simulink library "Contact_Forces_Lib"  (R2025b)
settings: Solver=ode45  StartTime=0.0  StopTime=10.0  RelTol=1e-3  EnableMultiTasking=on
undefined symbols (not defined in the file or in its folder): b_contact, custom_param_1, custom_param_2, Extr_Data_Ring, k_contact, l_cone, length_cylinder, length_tube, mu_kinetic, mu_static, pen_exponent, pen_full_damp_F, rad_s_cone, radius_cylinder, radius_tube, v_thr, X, Y, Z
libraries: nesl_utility x197, sm_lib x115, $bdroot x72, simulink x20, fl_lib x4
(part 7 of 12)

== system Contact_Forces_Lib/3D/Sphere in Sphere Force/Sensing ==
  Divide : Product  Inputs=*/
  Mux : Mux  Inputs=3
  Mux1 : Mux  Inputs=3
  Mux2 : Mux  Inputs=3
  PS-Simulink Converter{2..4,7..15} (12 alike) : nesl_utility/PS-Simulink Converter  PhysicalDomain=network_engine_domain  SubClassName=ps_output  LeftPortType=input  RightPortType=output  PseudoPeriodic=off  Frequencies=[]  VectorFormat=1-D array  Unit=1  AffineConversion=off
  Transform Sensor : sm_lib/Frames and Transforms/Transform Sensor  MeasurementFrame=Base  RotationSequence=XYX  SenseAngle=off  SenseAxis=off  SenseQ=off  SenseR=on  SenseRotationSequence=off  SenseOmegaX=on  SenseOmegaY=on  SenseOmegaZ=on  SenseOmega=off  SenseQDot=off  SenseRDot=off  SenseRotationSequenceDot=off  SenseAlphaX=off  SenseAlphaY=off  SenseAlphaZ=off  SenseAlpha=off  SenseQDDot=off  SenseRDDot=off  SenseX=on  SenseY=on  SenseZ=on  SenseXYZ=off  SenseRad=off  SenseAzim=off  SenseDist=on  SenseInc=off  SenseXDot=on  SenseYDot=on  SenseZDot=on  SenseXYZDot=off  SenseRadDot=off  SenseAzimDot=off  SenseDistDot=on  SenseIncDot=off  SenseXDDot=off  SenseYDDot=off  SenseZDDot=off  SenseXYZDDot=off  SenseRadDDot=off  SenseAzimDDot=off  SenseDistDDot=off  SenseIncDDot=off
  F : PMIOPort  Side=Left
  B : PMIOPort  Port=2  Side=Left
  R : Outport  VectorParamsAs1DForOutWhenUnconnected=off
  dst : Outport  Port=2  VectorParamsAs1DForOutWhenUnconnected=off
  vdst : Outport  Port=3  VectorParamsAs1DForOutWhenUnconnected=off
  dvect : Outport  Port=4  VectorParamsAs1DForOutWhenUnconnected=off
  v : Outport  Port=5  VectorParamsAs1DForOutWhenUnconnected=off
  w : Outport  Port=6  VectorParamsAs1DForOutWhenUnconnected=off
  wires:
  PS-Simulink Converter2/1 -> R/1
  PS-Simulink Converter7/1 -> Divide/2, dst/1
  PS-Simulink Converter8/1 -> vdst/1
  PS-Simulink Converter11/1 -> Mux/3
  PS-Simulink Converter10/1 -> Mux/2
  PS-Simulink Converter9/1 -> Mux/1
  Mux/1 -> Divide/1
  Divide/1 -> dvect/1
  PS-Simulink Converter3/1 -> Mux1/1
  PS-Simulink Converter4/1 -> Mux1/2
  PS-Simulink Converter12/1 -> Mux1/3
  Mux1/1 -> w/1
  PS-Simulink Converter14/1 -> Mux2/2
  PS-Simulink Converter15/1 -> Mux2/3
  PS-Simulink Converter13/1 -> Mux2/1
  Mux2/1 -> v/1
  connections:
  Transform Sensor/RConn1 -- F/RConn1
  Transform Sensor/LConn1 -- B/RConn1
  Transform Sensor/RConn2 -- PS-Simulink Converter2/LConn1
  Transform Sensor/RConn3 -- PS-Simulink Converter3/LConn1
  PS-Simulink Converter4/LConn1 -- Transform Sensor/RConn4
  PS-Simulink Converter8/LConn1 -- Transform Sensor/RConn13
  PS-Simulink Converter7/LConn1 -- Transform Sensor/RConn9
  Transform Sensor/RConn8 -- PS-Simulink Converter11/LConn1
  Transform Sensor/RConn7 -- PS-Simulink Converter10/LConn1
  Transform Sensor/RConn6 -- PS-Simulink Converter9/LConn1
  PS-Simulink Converter12/LConn1 -- Transform Sensor/RConn5
  PS-Simulink Converter13/LConn1 -- Transform Sensor/RConn10
  PS-Simulink Converter14/LConn1 -- Transform Sensor/RConn11
  PS-Simulink Converter15/LConn1 -- Transform Sensor/RConn12

== system Contact_Forces_Lib/3D/Sphere to Cone Force/Check Active ==
  z : Inport
  azm : Inport  Port=2
  Check Active Range : Subsystem
  Data Type Conversion : DataTypeConversion  SaturateOnIntegerOverflow=off  RndMeth=Floor
  In Tube : Subsystem
  Logical Operator : Logic  AllPortsSameDT=off  OutDataTypeStr=boolean
  En : Outport  VectorParamsAs1DForOutWhenUnconnected=off
  wires:
  Data Type Conversion/1 -> En/1
  In Tube/1(En) -> Logical Operator/1
  azm/1 -> Check Active Range/1(azm)
  z/1 -> In Tube/1(z)
  Check Active Range/1(En) -> Logical Operator/2
  Logical Operator/1 -> Data Type Conversion/1

== system Contact_Forces_Lib/3D/Sphere to Cone Force/Demux ==
  Frc : Inport
  Cone Forces : Scope  NumInputPorts=6
      settings: ActiveDisplayYMinimum=-7.50703109533E+6  ActiveDisplayYMaximum=872315.20608
  Demux : Demux  Outputs=8
  Demux1 : Demux  Outputs=3
  Demux2 : Demux  Outputs=3
  Simulink-PS Converter{,1..7} (8 alike) : nesl_utility/Simulink-PS Converter  PhysicalDomain=network_engine_domain  SubClassName=ps_input  LeftPortType=input  RightPortType=output  PseudoPeriodic=off  Frequencies=[]  NoiseDistribution=none  NoiseParameters=[]  Unit=1  AffineConversion=off  FilteringAndDerivatives=zero  SimscapeFilterOrder=1  InputFilterTimeConstant=0.005  UdotUserProvided=1
  Sphere Forces : Scope  NumInputPorts=6
      settings: ActiveDisplayYMinimum=-114928.22843  ActiveDisplayYMaximum=94591.09777
  FxF : PMIOPort  Side=Right
  FyF : PMIOPort  Port=2  Side=Right
  FzF : PMIOPort  Port=3  Side=Right
  TF : PMIOPort  Port=4  Side=Right
  FxB : PMIOPort  Port=5  Side=Right
  FyB : PMIOPort  Port=6  Side=Right
  FzB : PMIOPort  Port=7  Side=Right
  TB : PMIOPort  Port=8  Side=Right
  wires:
  Demux2/3 -> Cone Forces/6  "Tz"
  Demux2/2 -> Cone Forces/5  "Ty"
  Demux2/1 -> Cone Forces/4  "Tx"
  Demux1/3 -> Sphere Forces/6  "Tz"
  Demux1/2 -> Sphere Forces/5  "Ty"
  Demux1/1 -> Sphere Forces/4  "Tx"
  Frc/1 -> Demux/1
  Demux/1 -> Sphere Forces/1, Simulink-PS Converter/1  "Fx"
  Demux/2 -> Sphere Forces/2, Simulink-PS Converter1/1  "Fy"
  Demux/4 -> Simulink-PS Converter2/1, Demux1/1
  Demux/3 -> Simulink-PS Converter6/1, Sphere Forces/3  "Fz"
  Demux/8 -> Simulink-PS Converter5/1, Demux2/1
  Demux/5 -> Simulink-PS Converter3/1, Cone Forces/1  "Fx"
  Demux/6 -> Simulink-PS Converter4/1, Cone Forces/2  "Fy"
  Demux/7 -> Simulink-PS Converter7/1, Cone Forces/3  "Fz"
  connections:
  Simulink-PS Converter2/RConn1 -- TF/RConn1
  Simulink-PS Converter4/RConn1 -- FyB/RConn1
  Simulink-PS Converter3/RConn1 -- FxB/RConn1
  Simulink-PS Converter5/RConn1 -- TB/RConn1
  Simulink-PS Converter/RConn1 -- FxF/RConn1
  Simulink-PS Converter1/RConn1 -- FyF/RConn1
  Simulink-PS Converter6/RConn1 -- FzF/RConn1
  Simulink-PS Converter7/RConn1 -- FzB/RConn1

== system Contact_Forces_Lib/3D/Sphere to Cone Force/Forces ==
  z : Inport
  rad : Inport  Port=2
  vrad : Inport  Port=3
  azm : Inport  Port=4
  vazm : Inport  Port=5
  vzf : Inport  Port=6
  wzf : Inport  Port=7
  R : Inport  Port=8
  wxf : Inport  Port=9
  wyf : Inport  Port=10
  vazmx : Inport  Port=11
  vazmy : Inport  Port=12
  Action Port : ActionPort
  Bus Creator : BusCreator  Inputs=6
  Calculate Penetration : Subsystem
  Ff : Subsystem
  Fn : Subsystem
  Force Law : $bdroot/Force Law  SystemSampleTime=-1  LabelModeActiveChoice=Linear  VariantActivationTime=update diagram  EmptyChoice=off  PassThrough=off  PassThroughVariantControl=(default)  EmptyChoiceVariantControl=(default)  AllowFlexibleInterface=on  Latency=0  AutoFrameSizeCalculation=off
  Gain : Gain  Gain=-1
  Mux : Mux  Inputs=8
  Product : Product
  Sum : Subsystem
  Sum1 : Sum  Inputs=+-
  Frc : Outport  VectorParamsAs1DForOutWhenUnconnected=off
  Out : Outport  Port=2  InitialOutput=[0]  VectorParamsAs1DForOutWhenUnconnected=off
  wires:
  vazmy/1 -> Ff/14(vazmy)
  vazmx/1 -> Ff/13(vazmx)
  wyf/1 -> Ff/12(wyf)
  wxf/1 -> Ff/11(wxf)
  Gain/1 -> Ff/1(Fn)
  vazm/1 -> Ff/5(vazm)
  wzf/1 -> Ff/6(wzf)
  Fn/6(FzConB) -> Sum/6(FnzConB)
  Ff/8(TConB) -> Sum/16(TConB)
  Ff/7(TSphF) -> Sum/15(TzSphF)
  Ff/6(FzConB) -> Sum/14(FfzConB)
  Ff/5(FyConB) -> Sum/13(FfyConB)
  Ff/4(FxConB) -> Sum/12(FfxConB)
  Ff/3(FzSphF) -> Sum/11(FfzSphF)
  Ff/2(FySphF) -> Sum/10(FfySphF)
  Ff/1(FxSphF) -> Sum/9(FfxSphF)
  Fn/8(TyConB) -> Sum/8(TnyConB)
  Fn/7(TxConB) -> Sum/7(TnxConB)
  Fn/5(FyConB) -> Sum/5(FnyConB)
  Fn/4(FxConB) -> Sum/4(FnxConB)
  Fn/3(FZSphF) -> Sum/3(FnzSphF)
  Fn/1(FxSphF) -> Sum/1(FnxSphF)
  Fn/2(FySphF) -> Sum/2(FnySphF)
  z/1 -> Fn/2(z), Ff/2(z), Calculate Penetration/3(z)
  Bus Creator/1 -> Out/1
  Force Law/1 -> Bus Creator/4, Sum1/1  "Spr Force"
  Calculate Penetration/3(Pen Vel) -> Bus Creator/1, Force Law/2  "Penetration Vel"
  vrad/1 -> Calculate Penetration/2(vrad), Ff/9(vrad)
  rad/1 -> Calculate Penetration/1(rad), Ff/8(rad), Fn/3(rad)
  Product/1 -> Bus Creator/5, Gain/1, Fn/1(Fn)  "Normal Force"
  Calculate Penetration/2(Pen) -> Force Law/1, Ff/7(Pen), Bus Creator/2  "Penetration"
  Calculate Penetration/1(sign) -> Product/1
  Force Law/2 -> Bus Creator/3, Sum1/2  "Damp Force"
  Sum1/1 -> Product/2
  R/1 -> Fn/4(R), Ff/3(R)
  azm/1 -> Fn/5(azm), Ff/4(azm)
  Sum/2(FyF) -> Mux/2
  Sum/1(FxF) -> Mux/1
  Mux/1 -> Frc/1
  Sum/4(TzF) -> Mux/4
  Sum/5(FxB) -> Mux/5
  Sum/6(FyB) -> Mux/6
  Sum/3(FzF) -> Mux/3
  Ff/9(Ff) -> Bus Creator/6  "Friction Force"
  Sum/7(FzB) -> Mux/7
  Sum/8(TB) -> Mux/8
  vzf/1 -> Calculate Penetration/4(vzf), Ff/10(vzf)

== system Contact_Forces_Lib/3D/Sphere to Cone Force/No Force ==
  Action Port : ActionPort
  Zeros : Constant  Value=[0 0 0 0 0 0 0 0 0 0 0 0]  SampleTime=0
  F : Outport  InitialOutput=[0]  VectorParamsAs1DForOutWhenUnconnected=off
  wires:
  Zeros/1 -> F/1

== system Contact_Forces_Lib/3D/Sphere to Cone Force/Sensing ==
  PS-Simulink Converter{1..4,6..11} (10 alike) : nesl_utility/PS-Simulink Converter  PhysicalDomain=network_engine_domain  SubClassName=ps_output  LeftPortType=input  RightPortType=output  PseudoPeriodic=off  Frequencies=[]  VectorFormat=1-D array  Unit=1  AffineConversion=off
  Transform Sensor Base : sm_lib/Frames and Transforms/Transform Sensor  MeasurementFrame=Base  RotationSequence=XYX  SenseAngle=off  SenseAxis=off  SenseQ=off  SenseR=on  SenseRotationSequence=off  SenseOmegaX=on  SenseOmegaY=on  SenseOmegaZ=on  SenseOmega=off  SenseQDot=off  SenseRDot=off  SenseRotationSequenceDot=off  SenseAlphaX=off  SenseAlphaY=off  SenseAlphaZ=off  SenseAlpha=off  SenseQDDot=off  SenseRDDot=off  SenseX=on  SenseY=on  SenseZ=on  SenseXYZ=off  SenseRad=off  SenseAzim=off  SenseDist=off  SenseInc=off  SenseXDot=on  SenseYDot=on  SenseZDot=on  SenseXYZDot=off  SenseRadDot=off  SenseAzimDot=off  SenseDistDot=off  SenseIncDot=off  SenseXDDot=off  SenseYDDot=off  SenseZDDot=off  SenseXYZDDot=off  SenseRadDDot=off  SenseAzimDDot=off  SenseDistDDot=off  SenseIncDDot=off
  rad_azm_cal : Subsystem
  F : PMIOPort  Side=Left
  B : PMIOPort  Port=2  Side=Left
  z : Outport  VectorParamsAs1DForOutWhenUnconnected=off
  rad : Outport  Port=2  VectorParamsAs1DForOutWhenUnconnected=off
  vrad : Outport  Port=3  VectorParamsAs1DForOutWhenUnconnected=off
  azm : Outport  Port=4  VectorParamsAs1DForOutWhenUnconnected=off
  vazm : Outport  Port=5  VectorParamsAs1DForOutWhenUnconnected=off
  vzf : Outport  Port=6  VectorParamsAs1DForOutWhenUnconnected=off
  wzf : Outport  Port=7  VectorParamsAs1DForOutWhenUnconnected=off
  R : Outport  Port=8  VectorParamsAs1DForOutWhenUnconnected=off
  wxf : Outport  Port=9  VectorParamsAs1DForOutWhenUnconnected=off
  wyf : Outport  Port=10  VectorParamsAs1DForOutWhenUnconnected=off
  vazmx : Outport  Port=11  VectorParamsAs1DForOutWhenUnconnected=off
  vazmy : Outport  Port=12  VectorParamsAs1DForOutWhenUnconnected=off
  wires:
  rad_azm_cal/6(vazmy) -> vazmy/1
  rad_azm_cal/5(vazmx) -> vazmx/1
  PS-Simulink Converter7/1 -> z/1, rad_azm_cal/3(z)
  PS-Simulink Converter8/1 -> rad_azm_cal/1(x)
  PS-Simulink Converter9/1 -> rad_azm_cal/2(y)
  PS-Simulink Converter10/1 -> rad_azm_cal/4(vx)
  PS-Simulink Converter11/1 -> rad_azm_cal/5(vy)
  rad_azm_cal/1(rad) -> rad/1
  rad_azm_cal/2(azm) -> azm/1
  rad_azm_cal/3(radv) -> vrad/1
  rad_azm_cal/4(azmv) -> vazm/1
  PS-Simulink Converter6/1 -> R/1
  PS-Simulink Converter1/1 -> vzf/1, rad_azm_cal/6(vz)
  PS-Simulink Converter2/1 -> wzf/1
  PS-Simulink Converter3/1 -> wxf/1
  PS-Simulink Converter4/1 -> wyf/1
  connections:
  Transform Sensor Base/RConn1 -- F/RConn1
  Transform Sensor Base/LConn1 -- B/RConn1
  PS-Simulink Converter6/LConn1 -- Transform Sensor Base/RConn2
  PS-Simulink Converter3/LConn1 -- Transform Sensor Base/RConn3
  PS-Simulink Converter8/LConn1 -- Transform Sensor Base/RConn6
  Transform Sensor Base/RConn7 -- PS-Simulink Converter9/LConn1
  Transform Sensor Base/RConn8 -- PS-Simulink Converter7/LConn1
  Transform Sensor Base/RConn9 -- PS-Simulink Converter10/LConn1
  Transform Sensor Base/RConn10 -- PS-Simulink Converter11/LConn1
  Transform Sensor Base/RConn11 -- PS-Simulink Converter1/LConn1
  PS-Simulink Converter4/LConn1 -- Transform Sensor Base/RConn4
  PS-Simulink Converter2/LConn1 -- Transform Sensor Base/RConn5

== system Contact_Forces_Lib/3D/Sphere to Cone Force/Set Output ==
  Frc : Inport
  En : Inport  Port=2
  FrameSep : Inport  Port=3
  Bus Creator : BusCreator  Inputs=7
  Bus Selector : BusSelector  OutputSignals=Normal Force,Friction Force,Penetration,Penetration Vel,Spr Force,Damp Force
  Demux : Demux  Outputs=6
  Mux : Mux  Inputs=6
  Product : Product
  Out : Outport  VectorParamsAs1DForOutWhenUnconnected=off
  wires:
  Demux/3 -> Bus Creator/3  "Penetration"
  Demux/6 -> Bus Creator/6  "Damp Force"
  Demux/5 -> Bus Creator/5  "Spr Force"
  Demux/4 -> Bus Creator/4  "Penetration Vel"
  Demux/2 -> Bus Creator/2  "Friction Force"
  Demux/1 -> Bus Creator/1  "Normal Force"
  Product/1 -> Demux/1
  En/1 -> Product/1
  Mux/1 -> Product/2
  FrameSep/1 -> Bus Creator/7
  Frc/1 -> Bus Selector/1
  Bus Selector/5 -> Mux/5  "<Spr Force>"
  Bus Selector/1 -> Mux/1  "<Normal Force>"
  Bus Creator/1 -> Out/1
  Bus Selector/3 -> Mux/3  "<Penetration>"
  Bus Selector/6 -> Mux/6  "<Damp Force>"
  Bus Selector/4 -> Mux/4  "<Penetration Vel>"
  Bus Selector/2 -> Mux/2  "<Friction Force>"

== system Contact_Forces_Lib/3D/Sphere to Plane Force/Check Sphere on Plane ==
  x : Inport
  y : Inport  Port=2
  Abs : Abs  ZeroCross=off  SaturateOnIntegerOverflow=off
  Abs1 : Abs  ZeroCross=off  SaturateOnIntegerOverflow=off
  Check loc x-axis : simulink/Logic and Bit Operations/Compare To Constant  relop=<  const=plane_lenx  OutDataTypeStr=boolean  ZeroCross=off
  Check loc y-axis : simulink/Logic and Bit Operations/Compare To Constant  relop=<  const=plane_leny  OutDataTypeStr=boolean  ZeroCross=off
  Data Type Conversion : DataTypeConversion  SaturateOnIntegerOverflow=off  RndMeth=Floor
  Gain : Gain  Gain=2
  Gain1 : Gain  Gain=2
  Logical Operator : Logic  AllPortsSameDT=off  OutDataTypeStr=boolean
  En : Outport  VectorParamsAs1DForOutWhenUnconnected=off
  wires:
  Check loc x-axis/1 -> Logical Operator/1
  Logical Operator/1 -> Data Type Conversion/1
  y/1 -> Gain1/1
  Data Type Conversion/1 -> En/1
  x/1 -> Gain/1
  Gain/1 -> Abs/1
  Gain1/1 -> Abs1/1
  Abs/1 -> Check loc x-axis/1
  Abs1/1 -> Check loc y-axis/1
  Check loc y-axis/1 -> Logical Operator/2

== system Contact_Forces_Lib/3D/Sphere to Plane Force/Demux ==
  Frc : Inport
  Demux : Demux
  Simulink-PS Converter{,1..2,6} (4 alike) : nesl_utility/Simulink-PS Converter  PhysicalDomain=network_engine_domain  SubClassName=ps_input  LeftPortType=input  RightPortType=output  PseudoPeriodic=off  Frequencies=[]  NoiseDistribution=none  NoiseParameters=[]  Unit=1  AffineConversion=off  FilteringAndDerivatives=zero  SimscapeFilterOrder=1  InputFilterTimeConstant=0.005  UdotUserProvided=1
  FSph : PMIOPort  Side=Right
  TSph : PMIOPort  Port=2  Side=Right
  FPla : PMIOPort  Port=3  Side=Right
  TPla : PMIOPort  Port=4  Side=Right
  wires:
  Demux/3 -> Simulink-PS Converter6/1
  Demux/4 -> Simulink-PS Converter2/1
  Demux/2 -> Simulink-PS Converter1/1
  Demux/1 -> Simulink-PS Converter/1
  Frc/1 -> Demux/1
  connections:
  Simulink-PS Converter6/RConn1 -- FPla/RConn1
  Simulink-PS Converter1/RConn1 -- TSph/RConn1
  Simulink-PS Converter/RConn1 -- FSph/RConn1
  Simulink-PS Converter2/RConn1 -- TPla/RConn1

== system Contact_Forces_Lib/3D/Sphere to Plane Force/Enable Outputs ==
  Frc : Inport
  En : Inport  Port=2
  FrameSep : Inport  Port=3
  Bus Creator1 : BusCreator  Inputs=7
  Bus Selector : BusSelector  OutputSignals=Normal Force,Friction Force,Penetration,Penetration Vel,Spr Force,Damp Force
  Demux : Demux  Outputs=[1 3 1 1 1 1]
  Mux : Mux  Inputs=6
  Product : Product
  Out : Outport  VectorParamsAs1DForOutWhenUnconnected=off
  wires:
  Bus Selector/5 -> Mux/5  "<Spr Force>"
  Bus Selector/6 -> Mux/6  "<Damp Force>"
  Bus Selector/1 -> Mux/1  "<Normal Force>"
  FrameSep/1 -> Bus Creator1/7
  Bus Selector/4 -> Mux/4  "<Penetration Vel>"
  Frc/1 -> Bus Selector/1
  Bus Selector/2 -> Mux/2  "<Friction Force>"
  Bus Creator1/1 -> Out/1
  Bus Selector/3 -> Mux/3  "<Penetration>"
  Mux/1 -> Product/2
  En/1 -> Product/1
  Product/1 -> Demux/1
  Demux/3 -> Bus Creator1/3  "Penetration"
  Demux/5 -> Bus Creator1/5  "Spr Force"
  Demux/4 -> Bus Creator1/4  "Penetration Vel"
  Demux/6 -> Bus Creator1/6  "Damp Force"
  Demux/1 -> Bus Creator1/1  "Normal Force"
  Demux/2 -> Bus Creator1/2  "Friction Force"

== system Contact_Forces_Lib/3D/Sphere to Plane Force/Forces ==
  x : Inport
  y : Inport  Port=2
  z : Inport  Port=3
  vz : Inport  Port=4
  R : Inport  Port=5
  wx : Inport  Port=6
  wy : Inport  Port=7
  vx : Inport  Port=8
  vy : Inport  Port=9
  Action Port : ActionPort  ActionPortLabel=if { }
  Bus Creator : BusCreator  Inputs=6
  Calculate Penetration : Subsystem
  Copy for Merge : SignalConversion  OverrideOpt=off
  Cross Product : $bdroot/Math/Cross Product  SystemSampleTime=-1  VariantActivationTime=update diagram  EmptyChoice=off  PassThrough=off  PassThroughVariantControl=(default)  EmptyChoiceVariantControl=(default)  AllowFlexibleInterface=on  Latency=0  AutoFrameSizeCalculation=off
  Ff : Subsystem
  Fn : Subsystem
  Force Law : $bdroot/Force Law  SystemSampleTime=-1  LabelModeActiveChoice=Linear  VariantActivationTime=update diagram  EmptyChoice=off  PassThrough=off  PassThroughVariantControl=(default)  EmptyChoiceVariantControl=(default)  AllowFlexibleInterface=on  Latency=0  AutoFrameSizeCalculation=off
  Mux : Mux
  Mux2 : Mux  Inputs=3
  Product : Product
  Product1 : Product
  Sum : Sum
  Sum1 : Sum
  z1 : InportShadow  Port=3
  Frc : Outport  VectorParamsAs1DForOutWhenUnconnected=off
  Out : Outport  Port=2  VectorParamsAs1DForOutWhenUnconnected=off
  wires:
  Cross Product/1 -> Mux/4  "TPla"
  Ff/2(T Sph) -> Mux/2  "TSph"
  Sum/1 -> Mux/1  "FSph"
  wx/1 -> Ff/4(wx)
  wy/1 -> Ff/5(wy)
  vy/1 -> Ff/7(vy)
  Ff/3(Ff Pla) -> Bus Creator/6, Sum1/2  "Friction Force"
  x/1 -> Mux2/1
  z/1 -> Mux2/3
  y/1 -> Mux2/2
  Fn/1(Fn) -> Bus Creator/5  "Normal Force"
  Ff/1(Ff Sph) -> Sum/2
  Mux2/1 -> Cross Product/1
  Sum1/1 -> Cross Product/2, Copy for Merge/1  "FPla"
  Force Law/2 -> Product1/1
  R/1 -> Ff/2(R), Fn/1(R)
  Calculate Penetration/4(Vel Sign) -> Product1/2
  Calculate Penetration/1(Pos Sign) -> Product/1, Ff/3(zSign)
  Fn/3(FnB) -> Ff/1(Fn), Sum1/1
  Calculate Penetration/3(Pen Vel) -> Force Law/2, Bus Creator/2  "Penetration Vel"
  Calculate Penetration/2(Pen) -> Force Law/1, Bus Creator/1  "Penetration"
  z1/1 -> Calculate Penetration/1(z)
  vz/1 -> Calculate Penetration/2(vz)
  Force Law/1 -> Product/2
  Bus Creator/1 -> Out/1
  Mux/1 -> Frc/1
  Fn/2(FnF) -> Sum/1
  Product/1 -> Fn/2(SprF), Bus Creator/3  "Spr Force"
  Product1/1 -> Fn/3(DamF), Bus Creator/4  "Damp Force"
  vx/1 -> Ff/6(vx)
  Copy for Merge/1 -> Mux/3

== system Contact_Forces_Lib/3D/Sphere to Plane Force/No Force ==
  Action Port : ActionPort  ActionPortLabel=else { }
  Zeros : Constant  Value=[0 0 0 0 0 0 0 0 0 0 0 0]  SampleTime=0
  Frc : Outport  InitialOutput=[0 0 0 0 0 0 0 0 0 0 0 0]  VectorParamsAs1DForOutWhenUnconnected=off
  wires:
  Zeros/1 -> Frc/1

== system Contact_Forces_Lib/3D/Sphere to Plane Force/Sensing ==
  PS-Simulink Converter{,1..8} (9 alike) : nesl_utility/PS-Simulink Converter  PhysicalDomain=network_engine_domain  SubClassName=ps_output  LeftPortType=input  RightPortType=output  PseudoPeriodic=off  Frequencies=[]  VectorFormat=1-D array  Unit=1  AffineConversion=off
  Transform Sensor : sm_lib/Frames and Transforms/Transform Sensor  MeasurementFrame=Base  RotationSequence=XYX  SenseAngle=off  SenseAxis=off  SenseQ=off  SenseR=on  SenseRotationSequence=off  SenseOmegaX=on  SenseOmegaY=on  SenseOmegaZ=off  SenseOmega=off  SenseQDot=off  SenseRDot=off  SenseRotationSequenceDot=off  SenseAlphaX=off  SenseAlphaY=off  SenseAlphaZ=off  SenseAlpha=off  SenseQDDot=off  SenseRDDot=off  SenseX=on  SenseY=on  SenseZ=on  SenseXYZ=off  SenseRad=off  SenseAzim=off  SenseDist=off  SenseInc=off  SenseXDot=on  SenseYDot=on  SenseZDot=on  SenseXYZDot=off  SenseRadDot=off  SenseAzimDot=off  SenseDistDot=off  SenseIncDot=off  SenseXDDot=off  SenseYDDot=off  SenseZDDot=off  SenseXYZDDot=off  SenseRadDDot=off  SenseAzimDDot=off  SenseDistDDot=off  SenseIncDDot=off
  F : PMIOPort  Side=Left
  B : PMIOPort  Port=2  Side=Left
  x : Outport  VectorParamsAs1DForOutWhenUnconnected=off
  y : Outport  Port=2  VectorParamsAs1DForOutWhenUnconnected=off
  z : Outport  Port=3  VectorParamsAs1DForOutWhenUnconnected=off
  vz : Outport  Port=4  VectorParamsAs1DForOutWhenUnconnected=off
  R : Outport  Port=5  VectorParamsAs1DForOutWhenUnconnected=off
  wx : Outport  Port=6  VectorParamsAs1DForOutWhenUnconnected=off
  wy : Outport  Port=7  VectorParamsAs1DForOutWhenUnconnected=off
  vx : Outport  Port=8  VectorParamsAs1DForOutWhenUnconnected=off
  vy : Outport  Port=9  VectorParamsAs1DForOutWhenUnconnected=off
  wires:
  PS-Simulink Converter8/1 -> y/1
  PS-Simulink Converter7/1 -> x/1
  PS-Simulink Converter6/1 -> vy/1
  PS-Simulink Converter5/1 -> vx/1
  PS-Simulink Converter4/1 -> wy/1
  PS-Simulink Converter3/1 -> wx/1
  PS-Simulink Converter2/1 -> R/1
  PS-Simulink Converter/1 -> z/1
  PS-Simulink Converter1/1 -> vz/1
  connections:
  PS-Simulink Converter8/LConn1 -- Transform Sensor/RConn6
  PS-Simulink Converter7/LConn1 -- Transform Sensor/RConn5
  Transform Sensor/RConn7 -- PS-Simulink Converter/LConn1
  Transform Sensor/RConn8 -- PS-Simulink Converter5/LConn1
  Transform Sensor/RConn9 -- PS-Simulink Converter6/LConn1
  PS-Simulink Converter1/LConn1 -- Transform Sensor/RConn10
  PS-Simulink Converter4/LConn1 -- Transform Sensor/RConn4
  Transform Sensor/RConn3 -- PS-Simulink Converter3/LConn1
  Transform Sensor/RConn2 -- PS-Simulink Converter2/LConn1
  Transform Sensor/LConn1 -- B/RConn1
  Transform Sensor/RConn1 -- F/RConn1

== system Contact_Forces_Lib/3D/Sphere to Plane Force Enabled/Check Sphere on Plane ==
  x : Inport
  y : Inport  Port=2
  Abs : Abs  ZeroCross=off  SaturateOnIntegerOverflow=off
  Abs1 : Abs  ZeroCross=off  SaturateOnIntegerOverflow=off
  Check loc x-axis : simulink/Logic and Bit Operations/Compare To Constant  relop=<  const=plane_lenx  OutDataTypeStr=boolean  ZeroCross=off
  Check loc y-axis : simulink/Logic and Bit Operations/Compare To Constant  relop=<  const=plane_leny  OutDataTypeStr=boolean  ZeroCross=off
  Data Type Conversion : DataTypeConversion  SaturateOnIntegerOverflow=off  RndMeth=Floor
  Gain : Gain  Gain=2
  Gain1 : Gain  Gain=2
  Logical Operator : Logic  AllPortsSameDT=off  OutDataTypeStr=boolean
  En : Outport  VectorParamsAs1DForOutWhenUnconnected=off
  wires:
  Check loc y-axis/1 -> Logical Operator/2
  Abs1/1 -> Check loc y-axis/1
  Abs/1 -> Check loc x-axis/1
  Gain1/1 -> Abs1/1
  Gain/1 -> Abs/1
  x/1 -> Gain/1
  Data Type Conversion/1 -> En/1
  y/1 -> Gain1/1
  Logical Operator/1 -> Data Type Conversion/1
  Check loc x-axis/1 -> Logical Operator/1

== system Contact_Forces_Lib/3D/Sphere to Plane Force Enabled/Demux ==
  Frc : Inport
  Demux : Demux
  Simulink-PS Converter{,1..2,6} (4 alike) : nesl_utility/Simulink-PS Converter  PhysicalDomain=network_engine_domain  SubClassName=ps_input  LeftPortType=input  RightPortType=output  PseudoPeriodic=off  Frequencies=[]  NoiseDistribution=none  NoiseParameters=[]  Unit=1  AffineConversion=off  FilteringAndDerivatives=zero  SimscapeFilterOrder=1  InputFilterTimeConstant=0.005  UdotUserProvided=1
  FSph : PMIOPort  Side=Right
  TSph : PMIOPort  Port=2  Side=Right
  FPla : PMIOPort  Port=3  Side=Right
  TPla : PMIOPort  Port=4  Side=Right
  wires:
  Frc/1 -> Demux/1
  Demux/1 -> Simulink-PS Converter/1
  Demux/2 -> Simulink-PS Converter1/1
  Demux/4 -> Simulink-PS Converter2/1
  Demux/3 -> Simulink-PS Converter6/1
  connections:
  Simulink-PS Converter2/RConn1 -- TPla/RConn1
  Simulink-PS Converter/RConn1 -- FSph/RConn1
  Simulink-PS Converter1/RConn1 -- TSph/RConn1
  Simulink-PS Converter6/RConn1 -- FPla/RConn1

== system Contact_Forces_Lib/3D/Sphere to Plane Force Enabled/Enable Outputs ==
  Frc : Inport
  En : Inport  Port=2
  FrameSep : Inport  Port=3
  Bus Creator1 : BusCreator  Inputs=7
  Bus Selector : BusSelector  OutputSignals=Normal Force,Friction Force,Penetration,Penetration Vel,Spr Force,Damp Force
  Demux : Demux  Outputs=[1 3 1 1 1 1]
  Mux : Mux  Inputs=6
  Product : Product
  Out : Outport  VectorParamsAs1DForOutWhenUnconnected=off
  wires:
  Demux/2 -> Bus Creator1/2  "Friction Force"
  Demux/1 -> Bus Creator1/1  "Normal Force"
  Demux/6 -> Bus Creator1/6  "Damp Force"
  Demux/4 -> Bus Creator1/4  "Penetration Vel"
  Demux/5 -> Bus Creator1/5  "Spr Force"
  Demux/3 -> Bus Creator1/3  "Penetration"
  Product/1 -> Demux/1
  En/1 -> Product/1
  Mux/1 -> Product/2
  Bus Selector/3 -> Mux/3  "<Penetration>"
  Bus Creator1/1 -> Out/1
  Bus Selector/2 -> Mux/2  "<Friction Force>"
  Frc/1 -> Bus Selector/1
  Bus Selector/4 -> Mux/4  "<Penetration Vel>"
  FrameSep/1 -> Bus Creator1/7
  Bus Selector/1 -> Mux/1  "<Normal Force>"
  Bus Selector/6 -> Mux/6  "<Damp Force>"
  Bus Selector/5 -> Mux/5  "<Spr Force>"

== system Contact_Forces_Lib/3D/Sphere to Plane Force Enabled/Forces ==
  x : Inport
  y : Inport  Port=2
  z : Inport  Port=3
  vz : Inport  Port=4
  R : Inport  Port=5
  wx : Inport  Port=6
  wy : Inport  Port=7
  vx : Inport  Port=8
  vy : Inport  Port=9
  Action Port : ActionPort  ActionPortLabel=if { }
  Bus Creator : BusCreator  Inputs=6
  Calculate Penetration : Subsystem
  Copy for Merge : SignalConversion  OverrideOpt=off
  Cross Product : $bdroot/Math/Cross Product  SystemSampleTime=-1  VariantActivationTime=update diagram  EmptyChoice=off  PassThrough=off  PassThroughVariantControl=(default)  EmptyChoiceVariantControl=(default)  AllowFlexibleInterface=on  Latency=0  AutoFrameSizeCalculation=off
  Ff : Subsystem
  Fn : Subsystem
  Force Law : $bdroot/Force Law  SystemSampleTime=-1  LabelModeActiveChoice=Linear  VariantActivationTime=update diagram  EmptyChoice=off  PassThrough=off  PassThroughVariantControl=(default)  EmptyChoiceVariantControl=(default)  AllowFlexibleInterface=on  Latency=0  AutoFrameSizeCalculation=off
  Mux : Mux
  Mux2 : Mux  Inputs=3
  Product : Product
  Product1 : Product
  Sum : Sum
  Sum1 : Sum
  z1 : InportShadow  Port=3
  Frc : Outport  VectorParamsAs1DForOutWhenUnconnected=off
  Out : Outport  Port=2  VectorParamsAs1DForOutWhenUnconnected=off
  wires:
  Copy for Merge/1 -> Mux/3
  vx/1 -> Ff/6(vx)
  Product1/1 -> Bus Creator/4, Fn/3(DamF)  "Damp Force"
  Product/1 -> Bus Creator/3, Fn/2(SprF)  "Spr Force"
  Fn/2(FnF) -> Sum/1
  Mux/1 -> Frc/1
  Bus Creator/1 -> Out/1
  Force Law/1 -> Product/2
  vz/1 -> Calculate Penetration/2(vz)
  z1/1 -> Calculate Penetration/1(z)
  Calculate Penetration/2(Pen) -> Bus Creator/1, Force Law/1  "Penetration"
  Calculate Penetration/3(Pen Vel) -> Bus Creator/2, Force Law/2  "Penetration Vel"
  Fn/3(FnB) -> Sum1/1, Ff/1(Fn)
  Calculate Penetration/1(Pos Sign) -> Ff/3(zSign), Product/1
  Calculate Penetration/4(Vel Sign) -> Product1/2
  R/1 -> Fn/1(R), Ff/2(R)
  Force Law/2 -> Product1/1
  Sum1/1 -> Copy for Merge/1, Cross Product/2  "FPla"
  Mux2/1 -> Cross Product/1
  Ff/1(Ff Sph) -> Sum/2
  Fn/1(Fn) -> Bus Creator/5  "Normal Force"
  y/1 -> Mux2/2
  z/1 -> Mux2/3
  x/1 -> Mux2/1
  Ff/3(Ff Pla) -> Sum1/2, Bus Creator/6  "Friction Force"
  vy/1 -> Ff/7(vy)
  wy/1 -> Ff/5(wy)
  wx/1 -> Ff/4(wx)
  Sum/1 -> Mux/1  "FSph"
  Ff/2(T Sph) -> Mux/2  "TSph"
  Cross Product/1 -> Mux/4  "TPla"

== system Contact_Forces_Lib/3D/Sphere to Plane Force Enabled/No Force ==
  Action Port : ActionPort  ActionPortLabel=else { }
  Zeros : Constant  Value=[0 0 0 0 0 0 0 0 0 0 0 0]  SampleTime=0
  Frc : Outport  InitialOutput=[0 0 0 0 0 0 0 0 0 0 0 0]  VectorParamsAs1DForOutWhenUnconnected=off
  wires:
  Zeros/1 -> Frc/1

== system Contact_Forces_Lib/3D/Sphere to Plane Force Enabled/Sensing ==
  In : Inport
  Bus Selector : BusSelector  OutputSignals=vy,vx
  PS-Simulink Converter{,1..8} (9 alike) : nesl_utility/PS-Simulink Converter  PhysicalDomain=network_engine_domain  SubClassName=ps_output  LeftPortType=input  RightPortType=output  PseudoPeriodic=off  Frequencies=[]  VectorFormat=1-D array  Unit=1  AffineConversion=off
  Product : Product
  Product1 : Product
  Sign : Signum  ZeroCross=off
  Sum : Sum  Inputs=|+-
  Sum1 : Sum  Inputs=|+-
  Transform Sensor : sm_lib/Frames and Transforms/Transform Sensor  MeasurementFrame=Base  RotationSequence=XYX  SenseAngle=off  SenseAxis=off  SenseQ=off  SenseR=on  SenseRotationSequence=off  SenseOmegaX=on  SenseOmegaY=on  SenseOmegaZ=off  SenseOmega=off  SenseQDot=off  SenseRDot=off  SenseRotationSequenceDot=off  SenseAlphaX=off  SenseAlphaY=off  SenseAlphaZ=off  SenseAlpha=off  SenseQDDot=off  SenseRDDot=off  SenseX=on  SenseY=on  SenseZ=on  SenseXYZ=off  SenseRad=off  SenseAzim=off  SenseDist=off  SenseInc=off  SenseXDot=on  SenseYDot=on  SenseZDot=on  SenseXYZDot=off  SenseRadDot=off  SenseAzimDot=off  SenseDistDot=off  SenseIncDot=off  SenseXDDot=off  SenseYDDot=off  SenseZDDot=off  SenseXYZDDot=off  SenseRadDDot=off  SenseAzimDDot=off  SenseDistDDot=off  SenseIncDDot=off
  F : PMIOPort  Side=Left
  B : PMIOPort  Port=2  Side=Left
  x : Outport  VectorParamsAs1DForOutWhenUnconnected=off
  y : Outport  Port=2  VectorParamsAs1DForOutWhenUnconnected=off
  z : Outport  Port=3  VectorParamsAs1DForOutWhenUnconnected=off
  vz : Outport  Port=4  VectorParamsAs1DForOutWhenUnconnected=off
  R : Outport  Port=5  VectorParamsAs1DForOutWhenUnconnected=off
  wx : Outport  Port=6  VectorParamsAs1DForOutWhenUnconnected=off
  wy : Outport  Port=7  VectorParamsAs1DForOutWhenUnconnected=off
  vx : Outport  Port=8  VectorParamsAs1DForOutWhenUnconnected=off
  vy : Outport  Port=9  VectorParamsAs1DForOutWhenUnconnected=off
  wires:
  PS-Simulink Converter1/1 -> vz/1
  PS-Simulink Converter/1 -> Sign/1, z/1
  PS-Simulink Converter2/1 -> R/1
  PS-Simulink Converter3/1 -> wx/1
  PS-Simulink Converter4/1 -> wy/1
  PS-Simulink Converter7/1 -> x/1
  PS-Simulink Converter8/1 -> y/1
  PS-Simulink Converter5/1 -> Sum1/1
  In/1 -> Bus Selector/1
  Bus Selector/1 -> Product/2  "<vy>"
  Sign/1 -> Product1/2, Product/1
  Product/1 -> Sum/2
  PS-Simulink Converter6/1 -> Sum/1
  Sum/1 -> vy/1
  Sum1/1 -> vx/1
  Product1/1 -> Sum1/2
  Bus Selector/2 -> Product1/1  "<vx>"
  connections:
  Transform Sensor/RConn1 -- F/RConn1
  Transform Sensor/LConn1 -- B/RConn1
  Transform Sensor/RConn2 -- PS-Simulink Converter2/LConn1
  Transform Sensor/RConn3 -- PS-Simulink Converter3/LConn1
  PS-Simulink Converter4/LConn1 -- Transform Sensor/RConn4
  PS-Simulink Converter1/LConn1 -- Transform Sensor/RConn10
  Transform Sensor/RConn9 -- PS-Simulink Converter6/LConn1
  Transform Sensor/RConn8 -- PS-Simulink Converter5/LConn1
  Transform Sensor/RConn7 -- PS-Simulink Converter/LConn1
  PS-Simulink Converter7/LConn1 -- Transform Sensor/RConn5
  PS-Simulink Converter8/LConn1 -- Transform Sensor/RConn6

== system Contact_Forces_Lib/3D/Sphere to Sphere Force/Calculate Penetration ==
  dst : Inport
  vdst : Inport  Port=2
  Constant : Constant  Value=sphB_rad+sphF_rad
  Dead Zone : DeadZone  LowerValue=-inf  UpperValue=0
  Gain : Gain  Gain=-1
  Sum : Sum  Inputs=+-
  Pen : Outport  VectorParamsAs1DForOutWhenUnconnected=off
  Pen Vel : Outport  Port=2  VectorParamsAs1DForOutWhenUnconnected=off
  wires:
  Gain/1 -> Pen Vel/1
  Constant/1 -> Sum/1
  Sum/1 -> Dead Zone/1
  dst/1 -> Sum/2
  Dead Zone/1 -> Pen/1
  vdst/1 -> Gain/1

== system Contact_Forces_Lib/3D/Sphere to Sphere Force/Ff ==
  Fn : Inport
  R : Inport  Port=2
  dvect : Inport  Port=3
  v : Inport  Port=4
  w : Inport  Port=5
  Check w or v non zero : Subsystem
  Cross Product : $bdroot/Math/Cross Product  SystemSampleTime=-1  VariantActivationTime=update diagram  EmptyChoice=off  PassThrough=off  PassThroughVariantControl=(default)  EmptyChoiceVariantControl=(default)  AllowFlexibleInterface=on  Latency=0  AutoFrameSizeCalculation=off
  Cross Product1 : $bdroot/Math/Cross Product  SystemSampleTime=-1  VariantActivationTime=update diagram  EmptyChoice=off  PassThrough=off  PassThroughVariantControl=(default)  EmptyChoiceVariantControl=(default)  AllowFlexibleInterface=on  Latency=0  AutoFrameSizeCalculation=off
  Friction Law : $bdroot/Friction Law  SystemSampleTime=-1  LabelModeActiveChoice=Stick_Slip_C  VariantActivationTime=update diagram  EmptyChoice=off  PassThrough=off  PassThroughVariantControl=(default)  EmptyChoiceVariantControl=(default)  AllowFlexibleInterface=on  Latency=0  AutoFrameSizeCalculation=off
  Fx1 : Constant  Value=sphB_rad
  Fx2 : Constant  Value=sphF_rad
  Gain1 : Gain  Gain=-1
  Gain2 : Gain
  Gain3 : Gain  Gain=-1
  Merge : Merge
  Merge1 : Merge
  Product : Product
  Product1 : Product
  Product2 : Product  Inputs=/*  Multiplication=Matrix(*)
  Product3 : Product
  Product4 : Product  Inputs=/*  Multiplication=Matrix(*)
  SlipVel : Subsystem
  mag : Subsystem
  FSphF : Outport  VectorParamsAs1DForOutWhenUnconnected=off
  TSphF : Outport  Port=2  VectorParamsAs1DForOutWhenUnconnected=off
  FSphB : Outport  Port=3  VectorParamsAs1DForOutWhenUnconnected=off
  TSphB : Outport  Port=4  VectorParamsAs1DForOutWhenUnconnected=off
  Ff : Outport  Port=5  VectorParamsAs1DForOutWhenUnconnected=off
  wires:
  Merge1/1 -> Product3/2
  Merge/1 -> Friction Law/2
  SlipVel/2(vuvect) -> Merge1/1
  SlipVel/1(vabs) -> Merge/2
  Fn/1 -> mag/1(vect)
  mag/1(mag) -> Friction Law/1
  Friction Law/1 -> Ff/1, Product3/1
  w/1 -> SlipVel/1(w), Check w or v non zero/1(w)
  v/1 -> SlipVel/2(v), Check w or v non zero/2(v)
  Gain2/1 -> Product1/1
  Fx1/1 -> Product1/2
  Product1/1 -> Cross Product/1
  Cross Product/1 -> TSphB/1
  Product3/1 -> Cross Product/2, Gain1/1, FSphB/1
  Product2/1 -> TSphF/1
  Product/1 -> Cross Product1/1
  Gain3/1 -> Product/1
  Fx2/1 -> Product/2
  Gain1/1 -> Cross Product1/2, Product4/2
  dvect/1 -> SlipVel/3(dvect), Gain3/1, Gain2/1
  Cross Product1/1 -> Product2/2
  R/1 -> Product2/1, Product4/1
  Product4/1 -> FSphF/1
  Check w or v non zero/3(Use SlipVel) -> SlipVel/Action
  Check w or v non zero/1(else v is 0) -> Merge/1
  Check w or v non zero/2(else uv is 0) -> Merge1/2

== system Contact_Forces_Lib/3D/Sphere to Sphere Force/Fn ==
  R : Inport
  SprF : Inport  Port=2
  DamF : Inport  Port=3
  dvect : Inport  Port=4
  Gain : Gain  Gain=-1
  Product : Product
  Product2 : Product  Inputs=/*  Multiplication=Matrix(*)
  Sum : Sum  Inputs=|+-
  Fn : Outport  VectorParamsAs1DForOutWhenUnconnected=off
  FSphF : Outport  Port=2  VectorParamsAs1DForOutWhenUnconnected=off
  FSphB : Outport  Port=3  VectorParamsAs1DForOutWhenUnconnected=off
  wires:
  Product/1 -> Gain/1, Product2/2
  dvect/1 -> Product/1
  Sum/1 -> Product/2, Fn/1
  Product2/1 -> FSphF/1
  Gain/1 -> FSphB/1
  R/1 -> Product2/1
  DamF/1 -> Sum/2
  SprF/1 -> Sum/1

== system Contact_Forces_Lib/3D/Sphere to Sphere Force/Sensing ==
  Divide : Product  Inputs=*/
  Mux : Mux  Inputs=3
  Mux1 : Mux  Inputs=3
  Mux2 : Mux  Inputs=3
  PS-Simulink Converter{2..4,7..15} (12 alike) : nesl_utility/PS-Simulink Converter  PhysicalDomain=network_engine_domain  SubClassName=ps_output  LeftPortType=input  RightPortType=output  PseudoPeriodic=off  Frequencies=[]  VectorFormat=1-D array  Unit=1  AffineConversion=off
  Transform Sensor : sm_lib/Frames and Transforms/Transform Sensor  MeasurementFrame=Base  RotationSequence=XYX  SenseAngle=off  SenseAxis=off  SenseQ=off  SenseR=on  SenseRotationSequence=off  SenseOmegaX=on  SenseOmegaY=on  SenseOmegaZ=on  SenseOmega=off  SenseQDot=off  SenseRDot=off  SenseRotationSequenceDot=off  SenseAlphaX=off  SenseAlphaY=off  SenseAlphaZ=off  SenseAlpha=off  SenseQDDot=off  SenseRDDot=off  SenseX=on  SenseY=on  SenseZ=on  SenseXYZ=off  SenseRad=off  SenseAzim=off  SenseDist=on  SenseInc=off  SenseXDot=on  SenseYDot=on  SenseZDot=on  SenseXYZDot=off  SenseRadDot=off  SenseAzimDot=off  SenseDistDot=on  SenseIncDot=off  SenseXDDot=off  SenseYDDot=off  SenseZDDot=off  SenseXYZDDot=off  SenseRadDDot=off  SenseAzimDDot=off  SenseDistDDot=off  SenseIncDDot=off
  F : PMIOPort  Side=Left
  B : PMIOPort  Port=2  Side=Left
  R : Outport  VectorParamsAs1DForOutWhenUnconnected=off
  dst : Outport  Port=2  VectorParamsAs1DForOutWhenUnconnected=off
  vdst : Outport  Port=3  VectorParamsAs1DForOutWhenUnconnected=off
  dvect : Outport  Port=4  VectorParamsAs1DForOutWhenUnconnected=off
  v : Outport  Port=5  VectorParamsAs1DForOutWhenUnconnected=off
  w : Outport  Port=6  VectorParamsAs1DForOutWhenUnconnected=off
  wires:
  Mux2/1 -> v/1
  PS-Simulink Converter13/1 -> Mux2/1
  PS-Simulink Converter15/1 -> Mux2/3
  PS-Simulink Converter14/1 -> Mux2/2
  Mux1/1 -> w/1
  PS-Simulink Converter12/1 -> Mux1/3
  PS-Simulink Converter4/1 -> Mux1/2
  PS-Simulink Converter3/1 -> Mux1/1
  Divide/1 -> dvect/1
  Mux/1 -> Divide/1
  PS-Simulink Converter9/1 -> Mux/1
  PS-Simulink Converter10/1 -> Mux/2
  PS-Simulink Converter11/1 -> Mux/3
  PS-Simulink Converter8/1 -> vdst/1
  PS-Simulink Converter7/1 -> dst/1, Divide/2
  PS-Simulink Converter2/1 -> R/1
  connections:
  PS-Simulink Converter15/LConn1 -- Transform Sensor/RConn12
  PS-Simulink Converter14/LConn1 -- Transform Sensor/RConn11
  PS-Simulink Converter13/LConn1 -- Transform Sensor/RConn10
  PS-Simulink Converter12/LConn1 -- Transform Sensor/RConn5
  Transform Sensor/RConn6 -- PS-Simulink Converter9/LConn1
  Transform Sensor/RConn7 -- PS-Simulink Converter10/LConn1
  Transform Sensor/RConn8 -- PS-Simulink Converter11/LConn1
  PS-Simulink Converter7/LConn1 -- Transform Sensor/RConn9
  PS-Simulink Converter8/LConn1 -- Transform Sensor/RConn13
  PS-Simulink Converter4/LConn1 -- Transform Sensor/RConn4
  Transform Sensor/RConn3 -- PS-Simulink Converter3/LConn1
  Transform Sensor/RConn2 -- PS-Simulink Converter2/LConn1
  Transform Sensor/LConn1 -- B/RConn1
  Transform Sensor/RConn1 -- F/RConn1

== system Contact_Forces_Lib/3D/Sphere to Tube Force/Check Active ==
  z : Inport
  azm : Inport  Port=2
  Check Active Range : Subsystem
  Compare To Zero : simulink/Logic and Bit Operations/Compare To Zero  relop=>  OutDataTypeStr=boolean  ZeroCross=off
  Data Type Conversion : DataTypeConversion  SaturateOnIntegerOverflow=off  RndMeth=Floor
  In Tube : Subsystem
  Logical Operator : Logic  AllPortsSameDT=off  OutDataTypeStr=boolean
  En : Outport  VectorParamsAs1DForOutWhenUnconnected=off
  wires:
  Logical Operator/1 -> Data Type Conversion/1
  Check Active Range/1(En) -> Logical Operator/2
  In Tube/1(En) -> Compare To Zero/1
  z/1 -> In Tube/1(z)
  azm/1 -> Check Active Range/1(azm)
  Compare To Zero/1 -> Logical Operator/1
  Data Type Conversion/1 -> En/1

== system Contact_Forces_Lib/3D/Sphere to Tube Force/Demux ==
  Frc : Inport
  Demux : Demux  Outputs=8
  Demux1 : Demux  Outputs=3
  Scope : Scope  NumInputPorts=6
      settings: ActiveDisplayYMinimum=-242589.77791  ActiveDisplayYMaximum=277348.80714
  Simulink-PS Converter{,1..7} (8 alike) : nesl_utility/Simulink-PS Converter  PhysicalDomain=network_engine_domain  SubClassName=ps_input  LeftPortType=input  RightPortType=output  PseudoPeriodic=off  Frequencies=[]  NoiseDistribution=none  NoiseParameters=[]  Unit=1  AffineConversion=off  FilteringAndDerivatives=zero  SimscapeFilterOrder=1  InputFilterTimeConstant=0.005  UdotUserProvided=1
  FxF : PMIOPort  Side=Right
  FyF : PMIOPort  Port=2  Side=Right
  FzF : PMIOPort  Port=3  Side=Right
  TF : PMIOPort  Port=4  Side=Right
  FxB : PMIOPort  Port=5  Side=Right
  FyB : PMIOPort  Port=6  Side=Right
  FzB : PMIOPort  Port=7  Side=Right
  TB : PMIOPort  Port=8  Side=Right
  wires:
  Demux1/3 -> Scope/6  "Tz"
  Demux1/2 -> Scope/5  "Ty"
  Demux1/1 -> Scope/4  "Tx"
  Demux/5 -> Simulink-PS Converter3/1, Scope/1  "Fx"
  Demux/6 -> Simulink-PS Converter4/1, Scope/2  "Fy"
  Demux/8 -> Simulink-PS Converter5/1, Demux1/1
  Demux/7 -> Simulink-PS Converter7/1, Scope/3  "Fz"
  Demux/3 -> Simulink-PS Converter6/1  "Fz"
  Demux/4 -> Simulink-PS Converter2/1
  Demux/2 -> Simulink-PS Converter1/1  "Fy"
  Demux/1 -> Simulink-PS Converter/1  "Fx"
  Frc/1 -> Demux/1
  connections:
  Simulink-PS Converter7/RConn1 -- FzB/RConn1
  Simulink-PS Converter6/RConn1 -- FzF/RConn1
  Simulink-PS Converter1/RConn1 -- FyF/RConn1
  Simulink-PS Converter/RConn1 -- FxF/RConn1
  Simulink-PS Converter5/RConn1 -- TB/RConn1
  Simulink-PS Converter3/RConn1 -- FxB/RConn1
  Simulink-PS Converter4/RConn1 -- FyB/RConn1
  Simulink-PS Converter2/RConn1 -- TF/RConn1

== system Contact_Forces_Lib/3D/Sphere to Tube Force/Forces ==
  z : Inport
  rad : Inport  Port=2
  vrad : Inport  Port=3
  azm : Inport  Port=4
  vazm : Inport  Port=5
  wzf : Inport  Port=6
  R : Inport  Port=7
  vzf : Inport  Port=8
  wxf : Inport  Port=9
  wyf : Inport  Port=10
  Action Port : ActionPort
  Bus Creator : BusCreator  Inputs=6
  Calculate Penetration : Subsystem
  Ff : Subsystem
  Fn : Subsystem
  Force Law : $bdroot/Force Law  SystemSampleTime=-1  LabelModeActiveChoice=Linear  VariantActivationTime=update diagram  EmptyChoice=off  PassThrough=off  PassThroughVariantControl=(default)  EmptyChoiceVariantControl=(default)  AllowFlexibleInterface=on  Latency=0  AutoFrameSizeCalculation=off
  Gain : Gain  Gain=-1
  Mux : Mux  Inputs=8
  Product : Product
  Sum : Subsystem
  Sum1 : Sum  Inputs=+-
  Frc : Outport  VectorParamsAs1DForOutWhenUnconnected=off
  Out : Outport  Port=2  InitialOutput=[0]  VectorParamsAs1DForOutWhenUnconnected=off
  wires:
  wyf/1 -> Ff/11(wyf)
  wxf/1 -> Ff/10(wxf)
  Gain/1 -> Ff/1(Fn)
  vzf/1 -> Ff/9(vzf)
  wzf/1 -> Ff/6(wzf)
  vazm/1 -> Ff/5(vazm)
  Sum/8(TB) -> Mux/8
  Sum/7(FzB) -> Mux/7
  Ff/9(Ff) -> Bus Creator/6  "Friction Force"
  Sum/3(FzF) -> Mux/3
  Sum/6(FyB) -> Mux/6
  Sum/5(FxB) -> Mux/5
  Sum/4(TzF) -> Mux/4
  Mux/1 -> Frc/1
  Sum/1(FxF) -> Mux/1
  Sum/2(FyF) -> Mux/2
  azm/1 -> Ff/4(azm), Fn/4(azm)
  R/1 -> Ff/3(R), Fn/3(R)
  Sum1/1 -> Product/2
  Force Law/2 -> Sum1/2, Bus Creator/3  "Damp Force"
  Calculate Penetration/1(sign) -> Product/1
  Calculate Penetration/2(Pen) -> Force Law/1, Bus Creator/2, Ff/7(Pen)  "Penetration"
  Product/1 -> Gain/1, Fn/1(Fn), Bus Creator/5  "Normal Force"
  rad/1 -> Calculate Penetration/1(rad), Ff/8(rad)
  vrad/1 -> Calculate Penetration/2(vrad)
  Calculate Penetration/3(Pen Vel) -> Force Law/2, Bus Creator/1  "Penetration Vel"
  Force Law/1 -> Sum1/1, Bus Creator/4  "Spr Force"
  Bus Creator/1 -> Out/1
  z/1 -> Fn/2(z), Ff/2(z)
  Fn/2(FySphF) -> Sum/2(FnySphF)
  Fn/1(FxSphF) -> Sum/1(FnxSphF)
  Fn/3(FZSphF) -> Sum/3(FnzSphF)
  Fn/4(FxTubB) -> Sum/4(FnxTubB)
  Fn/5(FyTubB) -> Sum/5(FnyTubB)
  Fn/6(TxTubB) -> Sum/6(TnxTubB)
  Fn/7(TyTubB) -> Sum/7(TnyTubB)
  Ff/1(FxSphF) -> Sum/8(FfxSphF)
  Ff/2(FySohF) -> Sum/9(FfySphF)
  Ff/3(FzSphF) -> Sum/10(FfzSphF)
  Ff/4(FxTubB) -> Sum/11(FfxTubB)
  Ff/5(FyTubB) -> Sum/12(FfyTubB)
  Ff/6(FzTubB) -> Sum/13(FfzTubB)
  Ff/7(TSphF) -> Sum/14(TzSphF)
  Ff/8(TTubB) -> Sum/15(TTubB)

== system Contact_Forces_Lib/3D/Sphere to Tube Force/No Force ==
  Action Port : ActionPort
  Zeros : Constant  Value=[0 0 0 0 0 0 0 0 0 0 0 0]  SampleTime=0
  F : Outport  InitialOutput=[0]  VectorParamsAs1DForOutWhenUnconnected=off
  wires:
  Zeros/1 -> F/1

== system Contact_Forces_Lib/3D/Sphere to Tube Force/Sensing ==
  PS-Simulink Converter{1..4,6..11} (10 alike) : nesl_utility/PS-Simulink Converter  PhysicalDomain=network_engine_domain  SubClassName=ps_output  LeftPortType=input  RightPortType=output  PseudoPeriodic=off  Frequencies=[]  VectorFormat=1-D array  Unit=1  AffineConversion=off
  Transform Sensor Base : sm_lib/Frames and Transforms/Transform Sensor  MeasurementFrame=Base  RotationSequence=XYX  SenseAngle=off  SenseAxis=off  SenseQ=off  SenseR=on  SenseRotationSequence=off  SenseOmegaX=on  SenseOmegaY=on  SenseOmegaZ=on  SenseOmega=off  SenseQDot=off  SenseRDot=off  SenseRotationSequenceDot=off  SenseAlphaX=off  SenseAlphaY=off  SenseAlphaZ=off  SenseAlpha=off  SenseQDDot=off  SenseRDDot=off  SenseX=on  SenseY=on  SenseZ=on  SenseXYZ=off  SenseRad=off  SenseAzim=off  SenseDist=off  SenseInc=off  SenseXDot=on  SenseYDot=on  SenseZDot=on  SenseXYZDot=off  SenseRadDot=off  SenseAzimDot=off  SenseDistDot=off  SenseIncDot=off  SenseXDDot=off  SenseYDDot=off  SenseZDDot=off  SenseXYZDDot=off  SenseRadDDot=off  SenseAzimDDot=off  SenseDistDDot=off  SenseIncDDot=off
  rad_azm_cal : Subsystem
  F : PMIOPort  Side=Left
  B : PMIOPort  Port=2  Side=Left
  z : Outport  VectorParamsAs1DForOutWhenUnconnected=off
  rad : Outport  Port=2  VectorParamsAs1DForOutWhenUnconnected=off
  vrad : Outport  Port=3  VectorParamsAs1DForOutWhenUnconnected=off
  azm : Outport  Port=4  VectorParamsAs1DForOutWhenUnconnected=off
  vazm : Outport  Port=5  VectorParamsAs1DForOutWhenUnconnected=off
  wzf : Outport  Port=6  VectorParamsAs1DForOutWhenUnconnected=off
  R : Outport  Port=7  VectorParamsAs1DForOutWhenUnconnected=off
  vzf : Outport  Port=8  VectorParamsAs1DForOutWhenUnconnected=off
  wxf : Outport  Port=9  VectorParamsAs1DForOutWhenUnconnected=off
  wyf : Outport  Port=10  VectorParamsAs1DForOutWhenUnconnected=off
  wires:
  PS-Simulink Converter4/1 -> wyf/1
  PS-Simulink Converter3/1 -> wxf/1
  PS-Simulink Converter2/1 -> wzf/1
  PS-Simulink Converter1/1 -> vzf/1
  PS-Simulink Converter6/1 -> R/1
  rad_azm_cal/4(azmv) -> vazm/1
  rad_azm_cal/3(radv) -> vrad/1
  rad_azm_cal/2(azm) -> azm/1
  rad_azm_cal/1(rad) -> rad/1
  PS-Simulink Converter11/1 -> rad_azm_cal/4(Ydot)
  PS-Simulink Converter10/1 -> rad_azm_cal/3(Xdot)
  PS-Simulink Converter9/1 -> rad_azm_cal/2(Y)
  PS-Simulink Converter8/1 -> rad_azm_cal/1(X)
  PS-Simulink Converter7/1 -> z/1
  connections:
  PS-Simulink Converter2/LConn1 -- Transform Sensor Base/RConn5
  PS-Simulink Converter4/LConn1 -- Transform Sensor Base/RConn4
  Transform Sensor Base/RConn11 -- PS-Simulink Converter1/LConn1
  Transform Sensor Base/RConn10 -- PS-Simulink Converter11/LConn1
  Transform Sensor Base/RConn9 -- PS-Simulink Converter10/LConn1
  Transform Sensor Base/RConn8 -- PS-Simulink Converter7/LConn1
  Transform Sensor Base/RConn7 -- PS-Simulink Converter9/LConn1
  PS-Simulink Converter8/LConn1 -- Transform Sensor Base/RConn6
  PS-Simulink Converter3/LConn1 -- Transform Sensor Base/RConn3
  PS-Simulink Converter6/LConn1 -- Transform Sensor Base/RConn2
  Transform Sensor Base/LConn1 -- B/RConn1
  Transform Sensor Base/RConn1 -- F/RConn1

== system Contact_Forces_Lib/3D/Sphere to Tube Force/Set Output ==
  Frc : Inport
  En : Inport  Port=2
  FrameSep : Inport  Port=3
  Bus Creator : BusCreator  Inputs=7
  Bus Selector : BusSelector  OutputSignals=Normal Force,Friction Force,Penetration,Penetration Vel,Spr Force,Damp Force
  Demux : Demux  Outputs=6
  Mux : Mux  Inputs=6
  Product : Product
  Out : Outport  VectorParamsAs1DForOutWhenUnconnected=off
  wires:
  Bus Selector/2 -> Mux/2  "<Friction Force>"
  Bus Selector/4 -> Mux/4  "<Penetration Vel>"
  Bus Selector/6 -> Mux/6  "<Damp Force>"
  Bus Selector/3 -> Mux/3  "<Penetration>"
  Bus Creator/1 -> Out/1
  Bus Selector/1 -> Mux/1  "<Normal Force>"
  Bus Selector/5 -> Mux/5  "<Spr Force>"
  Frc/1 -> Bus Selector/1
  FrameSep/1 -> Bus Creator/7
  Mux/1 -> Product/2
  En/1 -> Product/1
  Product/1 -> Demux/1
  Demux/1 -> Bus Creator/1  "Normal Force"
  Demux/2 -> Bus Creator/2  "Friction Force"
  Demux/4 -> Bus Creator/4  "Penetration Vel"
  Demux/5 -> Bus Creator/5  "Spr Force"
  Demux/6 -> Bus Creator/6  "Damp Force"
  Demux/3 -> Bus Creator/3  "Penetration"

== system Contact_Forces_Lib/3D/Sphere to Tube Force Enabled/Check Active ==
  z : Inport
  azm : Inport  Port=2
  Check Active Range : Subsystem
  Compare To Zero : simulink/Logic and Bit Operations/Compare To Zero  relop=>  OutDataTypeStr=boolean  ZeroCross=off
  Data Type Conversion : DataTypeConversion  SaturateOnIntegerOverflow=off  RndMeth=Floor
  In Tube : Subsystem
  Logical Operator : Logic  AllPortsSameDT=off  OutDataTypeStr=boolean
  En : Outport  VectorParamsAs1DForOutWhenUnconnected=off
  wires:
  Logical Operator/1 -> Data Type Conversion/1
  Check Active Range/1(En) -> Logical Operator/2
  In Tube/1(En) -> Compare To Zero/1
  z/1 -> In Tube/1(z)
  azm/1 -> Check Active Range/1(azm)
  Compare To Zero/1 -> Logical Operator/1
  Data Type Conversion/1 -> En/1
